simulink model "servo_20230915"  (R2022a)
settings: Solver=ode45  StartTime=0.0  StopTime=5  RelTol=1e-3
model workspace (MAT data in the model file):
  J = 0.0095
  Kt = 1
  La = 0.00097
  Ra = 0.11
values from neighbouring files (symbols this model uses):
  fe = 0.008    [para_for_math_pmsm.m]
  flux = 0.1827    [para_for_math_pmsm.m]
  Je = 0.003    [para_for_math_pmsm.m]
  Ld = 5.25e-3    (= 0.00525)    [para_for_math_pmsm.m]
  Lq = 5.25e-3    (= 0.00525)    [para_for_math_pmsm.m]
  Pn = 4    [para_for_math_pmsm.m]
  R = 0.299    [init_dc_servo.m]    (also in para_for_math_pmsm.m = 0.958)
undefined symbols (not defined in the file or in its folder): smiData, X, Y, Z
libraries: sm_lib x30, nesl_utility x16, spspowerguiLib x1
settings Model: ParameterArgumentNames=La,Ra  Creator=ccaao  LastModifiedBy=ccaao

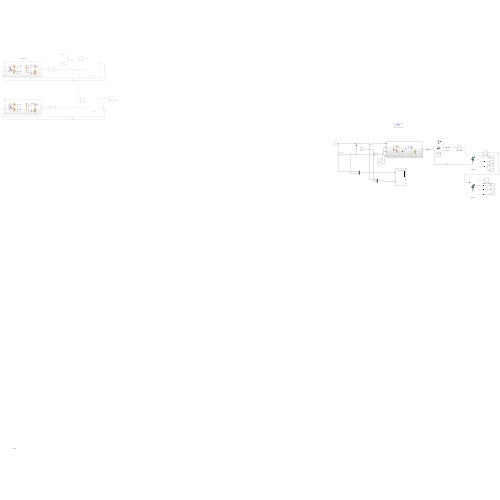
[thumbnail: Simulink's stored preview of the top-level diagram]
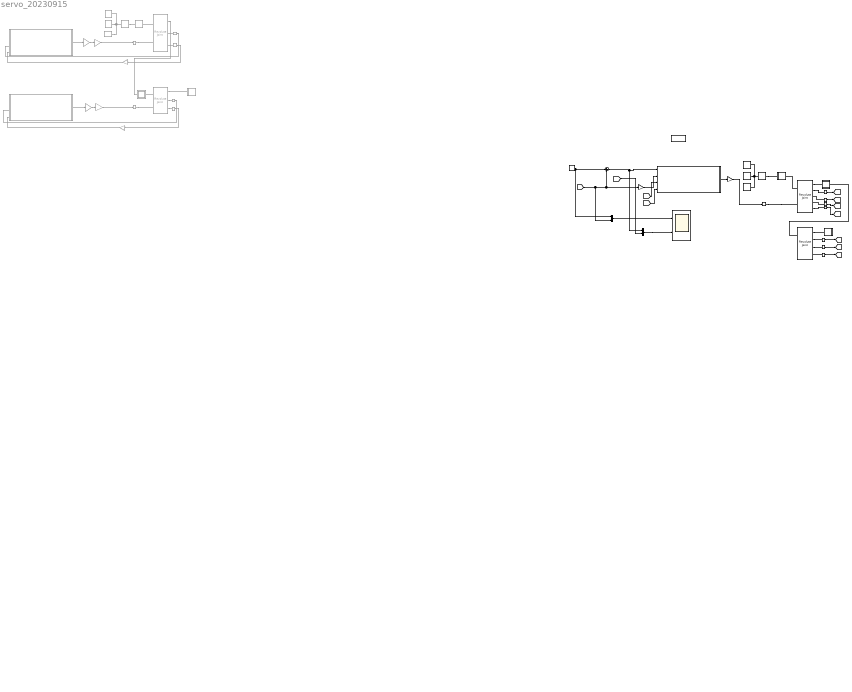
== system servo_20230915 ==
  note: position
  note: 电机方程
  Constant : Constant  Value=10
  Gain : Gain  Commented=on
  Gain1 : Gain  Commented=on  Gain=0.95
  Gain2 : Gain  Commented=on
  Gain3 : Gain  Commented=on  Gain=0.95
  Gain4 : Gain  Commented=on  Gain=Pn
  Gain5 : Gain  Commented=on  Gain=Pn
  Gain6 : Gain  Gain=Pn
  Gain8 : Gain  Gain=0.95
  MechanismConfiguration : sm_lib/Utilities/Mechanism Configuration  Commented=on  UniformGravity=Constant  GravityVector=[0 -9.80665 0]  GravityUnits=m/s^2  LinearizationDelta=0.001  JointModeTransitionNonlinearIterations=2
  MechanismConfiguration1 : sm_lib/Utilities/Mechanism Configuration  UniformGravity=Constant  GravityVector=[0 0 0]  GravityUnits=m/s^2  LinearizationDelta=0.001  JointModeTransitionNonlinearIterations=2
  Mux : Mux  Inputs=2
  Mux1 : Mux  Inputs=2
  PS-Simulink Converter{,1..3} (4 alike) : nesl_utility/PS-Simulink Converter  Commented=on  PhysicalDomain=network_engine_domain  SubClassName=ps_output  LeftPortType=input  RightPortType=output  PseudoPeriodic=off  Frequencies=[]  VectorFormat=inherit  Unit=inherit  AffineConversion=off
      settings: SourceProductBaseCode=SS,PW,VE
  PS-Simulink Converter10 : nesl_utility/PS-Simulink Converter  PhysicalDomain=network_engine_domain  SubClassName=ps_output  LeftPortType=input  RightPortType=output  PseudoPeriodic=off  Frequencies=[]  VectorFormat=1-D array  Unit=inherit  AffineConversion=off
      settings: SourceProductBaseCode=SS,PW,VE
  PS-Simulink Converter4 : nesl_utility/PS-Simulink Converter  PhysicalDomain=network_engine_domain  SubClassName=ps_output  LeftPortType=input  RightPortType=output  PseudoPeriodic=off  Frequencies=[]  VectorFormat=1-D array  Unit=rad  AffineConversion=off
      settings: SourceProductBaseCode=SS,PW,VE
  PS-Simulink Converter5 : nesl_utility/PS-Simulink Converter  PhysicalDomain=network_engine_domain  SubClassName=ps_output  LeftPortType=input  RightPortType=output  PseudoPeriodic=off  Frequencies=[]  VectorFormat=1-D array  Unit=N*m  AffineConversion=off
      settings: SourceProductBaseCode=SS,PW,VE
  PS-Simulink Converter6 : nesl_utility/PS-Simulink Converter  PhysicalDomain=network_engine_domain  SubClassName=ps_output  LeftPortType=input  RightPortType=output  PseudoPeriodic=off  Frequencies=[]  VectorFormat=1-D array  Unit=rad/s  AffineConversion=off
      settings: SourceProductBaseCode=SS,PW,VE
  PS-Simulink Converter7 : nesl_utility/PS-Simulink Converter  PhysicalDomain=network_engine_domain  SubClassName=ps_output  LeftPortType=input  RightPortType=output  PseudoPeriodic=off  Frequencies=[]  VectorFormat=1-D array  Unit=N*m  AffineConversion=off
      settings: SourceProductBaseCode=SS,PW,VE
  PS-Simulink Converter8 : nesl_utility/PS-Simulink Converter  PhysicalDomain=network_engine_domain  SubClassName=ps_output  LeftPortType=input  RightPortType=output  PseudoPeriodic=off  Frequencies=[]  VectorFormat=1-D array  Unit=rad  AffineConversion=off
      settings: SourceProductBaseCode=SS,PW,VE
  PS-Simulink Converter9 : nesl_utility/PS-Simulink Converter  PhysicalDomain=network_engine_domain  SubClassName=ps_output  LeftPortType=input  RightPortType=output  PseudoPeriodic=off  Frequencies=[]  VectorFormat=1-D array  Unit=rad/s  AffineConversion=off
      settings: SourceProductBaseCode=SS,PW,VE
  Revolute : sm_lib/Joints/Revolute Joint  Commented=on  JointMode=Normal  SenseConstraintForce=off  SenseConstraintForceX=off  SenseConstraintForceY=off  SenseConstraintForceZ=off  SenseConstraintTorque=off  SenseConstraintTorqueX=off  SenseConstraintTorqueY=off  SenseConstraintTorqueZ=off  SenseTotalForce=off  SenseTotalForceX=off  SenseTotalForceY=off  SenseTotalForceZ=off  SenseTotalTorque=off  SenseTotalTorqueX=off  SenseTotalTorqueY=off  SenseTotalTorqueZ=off  CompositeWrenchDir=FollowerOnBase  CompositeWrenchFrame=BaseFrame  EquilibriumPosition=0  EquilibriumPositionUnits=rad  SpringStiffness=0  SpringStiffnessUnits=N*m/rad  DampingCoefficient=0  DampingCoefficientUnits=N*m/(rad/s)  TorqueActuationMode=InputTorque  MotionActuationMode=ComputedMotion  SensePosition=on  SenseVelocity=on  SenseAcceleration=off  SenseTorqueForce=off  SenseLowerLimitTorqueForce=off  SenseUpperLimitTorqueForce=off  LowerLimitSpecify=off  LowerLimitBound=-90  LowerLimitBoundUnits=deg  LowerLimitStiffness=1e4  LowerLimitStiffnessUnits=N*m/deg  LowerLimitDamping=10  LowerLimitDampingUnits=N*m/(deg/s)  LowerLimitTransitionRegionWidth=0.1  LowerLimitTransitionRegionWidthUnits=deg  UpperLimitSpecify=off  UpperLimitBound=90  UpperLimitBoundUnits=deg  UpperLimitStiffness=1e4  UpperLimitStiffnessUnits=N*m/deg  UpperLimitDamping=10  UpperLimitDampingUnits=N*m/(deg/s)  UpperLimitTransitionRegionWidth=0.1  UpperLimitTransitionRegionWidthUnits=deg  PositionTargetSpecify=on  PositionTargetPriority=High  PositionTargetValue=smiData.RevoluteJoint(1).Rz.Pos  PositionTargetValueUnits=deg  VelocityTargetSpecify=on  VelocityTargetPriority=High  VelocityTargetValue=0  VelocityTargetValueUnits=rad/s
  Revolute1 : sm_lib/Joints/Revolute Joint  Commented=on  JointMode=Normal  SenseConstraintForce=off  SenseConstraintForceX=off  SenseConstraintForceY=off  SenseConstraintForceZ=off  SenseConstraintTorque=off  SenseConstraintTorqueX=off  SenseConstraintTorqueY=off  SenseConstraintTorqueZ=off  SenseTotalForce=off  SenseTotalForceX=off  SenseTotalForceY=off  SenseTotalForceZ=off  SenseTotalTorque=off  SenseTotalTorqueX=off  SenseTotalTorqueY=off  SenseTotalTorqueZ=off  CompositeWrenchDir=FollowerOnBase  CompositeWrenchFrame=BaseFrame  EquilibriumPosition=0  EquilibriumPositionUnits=rad  SpringStiffness=0  SpringStiffnessUnits=N*m/rad  DampingCoefficient=0  DampingCoefficientUnits=N*m/(rad/s)  TorqueActuationMode=InputTorque  MotionActuationMode=ComputedMotion  SensePosition=on  SenseVelocity=on  SenseAcceleration=off  SenseTorqueForce=off  SenseLowerLimitTorqueForce=off  SenseUpperLimitTorqueForce=off  LowerLimitSpecify=off  LowerLimitBound=-90  LowerLimitBoundUnits=deg  LowerLimitStiffness=1e4  LowerLimitStiffnessUnits=N*m/deg  LowerLimitDamping=10  LowerLimitDampingUnits=N*m/(deg/s)  LowerLimitTransitionRegionWidth=0.1  LowerLimitTransitionRegionWidthUnits=deg  UpperLimitSpecify=off  UpperLimitBound=90  UpperLimitBoundUnits=deg  UpperLimitStiffness=1e4  UpperLimitStiffnessUnits=N*m/deg  UpperLimitDamping=10  UpperLimitDampingUnits=N*m/(deg/s)  UpperLimitTransitionRegionWidth=0.1  UpperLimitTransitionRegionWidthUnits=deg  PositionTargetSpecify=on  PositionTargetPriority=High  PositionTargetValue=smiData.RevoluteJoint(2).Rz.Pos  PositionTargetValueUnits=deg  VelocityTargetSpecify=on  VelocityTargetPriority=High  VelocityTargetValue=0  VelocityTargetValueUnits=rad/s
  Revolute2 : sm_lib/Joints/Revolute Joint  JointMode=Normal  SenseConstraintForce=off  SenseConstraintForceX=off  SenseConstraintForceY=off  SenseConstraintForceZ=off  SenseConstraintTorque=off  SenseConstraintTorqueX=off  SenseConstraintTorqueY=off  SenseConstraintTorqueZ=off  SenseTotalForce=off  SenseTotalForceX=off  SenseTotalForceY=off  SenseTotalForceZ=off  SenseTotalTorque=off  SenseTotalTorqueX=off  SenseTotalTorqueY=off  SenseTotalTorqueZ=off  CompositeWrenchDir=FollowerOnBase  CompositeWrenchFrame=BaseFrame  EquilibriumPosition=0  EquilibriumPositionUnits=rad  SpringStiffness=0  SpringStiffnessUnits=N*m/rad  DampingCoefficient=0.0001  DampingCoefficientUnits=N*m/(rad/s)  TorqueActuationMode=InputTorque  MotionActuationMode=ComputedMotion  SensePosition=on  SenseVelocity=on  SenseAcceleration=on  SenseTorqueForce=on  SenseLowerLimitTorqueForce=off  SenseUpperLimitTorqueForce=off  LowerLimitSpecify=off  LowerLimitBound=-90  LowerLimitBoundUnits=deg  LowerLimitStiffness=1e4  LowerLimitStiffnessUnits=N*m/deg  LowerLimitDamping=10  LowerLimitDampingUnits=N*m/(deg/s)  LowerLimitTransitionRegionWidth=0.1  LowerLimitTransitionRegionWidthUnits=deg  UpperLimitSpecify=off  UpperLimitBound=90  UpperLimitBoundUnits=deg  UpperLimitStiffness=1e4  UpperLimitStiffnessUnits=N*m/deg  UpperLimitDamping=10  UpperLimitDampingUnits=N*m/(deg/s)  UpperLimitTransitionRegionWidth=0.1  UpperLimitTransitionRegionWidthUnits=deg  PositionTargetSpecify=off  PositionTargetPriority=High  PositionTargetValue=smiData.RevoluteJoint(1).Rz.Pos  PositionTargetValueUnits=deg  VelocityTargetSpecify=on  VelocityTargetPriority=High  VelocityTargetValue=0  VelocityTargetValueUnits=rad/s
  Revolute3 : sm_lib/Joints/Revolute Joint  JointMode=Normal  SenseConstraintForce=off  SenseConstraintForceX=off  SenseConstraintForceY=off  SenseConstraintForceZ=off  SenseConstraintTorque=off  SenseConstraintTorqueX=off  SenseConstraintTorqueY=off  SenseConstraintTorqueZ=off  SenseTotalForce=off  SenseTotalForceX=off  SenseTotalForceY=off  SenseTotalForceZ=off  SenseTotalTorque=off  SenseTotalTorqueX=off  SenseTotalTorqueY=off  SenseTotalTorqueZ=off  CompositeWrenchDir=FollowerOnBase  CompositeWrenchFrame=BaseFrame  EquilibriumPosition=0  EquilibriumPositionUnits=rad  SpringStiffness=1000  SpringStiffnessUnits=N*m/rad  DampingCoefficient=0.0001  DampingCoefficientUnits=N*m/(rad/s)  TorqueActuationMode=InputTorque  MotionActuationMode=ComputedMotion  SensePosition=on  SenseVelocity=on  SenseAcceleration=off  SenseTorqueForce=on  SenseLowerLimitTorqueForce=off  SenseUpperLimitTorqueForce=off  LowerLimitSpecify=on  LowerLimitBound=40  LowerLimitBoundUnits=deg  LowerLimitStiffness=1e7  LowerLimitStiffnessUnits=N*m/deg  LowerLimitDamping=10  LowerLimitDampingUnits=N*m/(deg/s)  LowerLimitTransitionRegionWidth=100  LowerLimitTransitionRegionWidthUnits=deg  UpperLimitSpecify=on  UpperLimitBound=120  UpperLimitBoundUnits=deg  UpperLimitStiffness=1e7  UpperLimitStiffnessUnits=N*m/deg  UpperLimitDamping=10  UpperLimitDampingUnits=N*m/(deg/s)  UpperLimitTransitionRegionWidth=100  UpperLimitTransitionRegionWidthUnits=deg  PositionTargetSpecify=on  PositionTargetPriority=Low  PositionTargetValue=80  PositionTargetValueUnits=deg  VelocityTargetSpecify=on  VelocityTargetPriority=High  VelocityTargetValue=0  VelocityTargetValueUnits=rad/s
  Scope : Scope  NumInputPorts=2
  Simulink-PS Converter : nesl_utility/Simulink-PS Converter  Commented=on  PhysicalDomain=network_engine_domain  SubClassName=ps_input  LeftPortType=input  RightPortType=output  PseudoPeriodic=off  Frequencies=[]  NoiseDistribution=none  NoiseParameters=[]  Unit=1  AffineConversion=off  FilteringAndDerivatives=provide  SimscapeFilterOrder=1  InputFilterTimeConstant=0.001  UdotUserProvided=0
      settings: SourceProductBaseCode=SS,PW,VE
  Simulink-PS Converter1 : nesl_utility/Simulink-PS Converter  Commented=on  PhysicalDomain=network_engine_domain  SubClassName=ps_input  LeftPortType=input  RightPortType=output  PseudoPeriodic=off  Frequencies=[]  NoiseDistribution=none  NoiseParameters=[]  Unit=1  AffineConversion=off  FilteringAndDerivatives=provide  SimscapeFilterOrder=1  InputFilterTimeConstant=0.001  UdotUserProvided=0
      settings: SourceProductBaseCode=SS,PW,VE
  Simulink-PS Converter2 : nesl_utility/Simulink-PS Converter  PhysicalDomain=network_engine_domain  SubClassName=ps_input  LeftPortType=input  RightPortType=output  PseudoPeriodic=off  Frequencies=[]  NoiseDistribution=none  NoiseParameters=[]  Unit=1  AffineConversion=off  FilteringAndDerivatives=provide  SimscapeFilterOrder=1  InputFilterTimeConstant=0.001  UdotUserProvided=0
      settings: SourceProductBaseCode=SS,PW,VE
  Solver Configuration : nesl_utility/Solver Configuration  Commented=on  PhysicalDomain=network_engine_domain  SubClassName=solver  LeftPortType=input  RightPortType=generic  Tones=[]  Harmonics=[]  SimulateNoise=off  Profile=off  UseLocalSampling=off  EnableSwitchedLinearOptims=on  FrequencyDomain=off  UseCCode=off  RelTol=0.001  AbsTol=0.001  MinStep=1e-09  ToWorkspace=off  RevertToSquareIcSolve=off  NumHomotopyIterations=100  PhasorMode=off  PhasorModeNumHarmonics=1  IndexReductionMethod=DerivativeReplacement  DoDC=off  ResidualTolerance=1e-09  UseLocalSolver=off  LocalSolverChoice=NE_BACKWARD_EULER_ADVANCER  LocalSolverSampleTime=0.001  DoFixedCost=off  MaxNonlinIter=3  MaxModeIter=2  ComputeImpulses=off  ImpulseIterations=2  LinearAlgebra=auto  LinearAlgebraNumThread=0  EquationFormulation=NE_TIME_EF  DelaysMemoryBudget=1024  AutomaticFiltering=on  FilteringTimeConstant=0.001  PartitionStorageMethod=AS_NEEDED  PartitionMemoryBudget=1024  PartitionMethod=ROBUST
      settings: SourceProductBaseCode=SS,PW,VE
  Solver Configuration1 : nesl_utility/Solver Configuration  PhysicalDomain=network_engine_domain  SubClassName=solver  LeftPortType=input  RightPortType=generic  Tones=[]  Harmonics=[]  SimulateNoise=off  Profile=off  UseLocalSampling=off  EnableSwitchedLinearOptims=on  FrequencyDomain=off  UseCCode=off  RelTol=0.001  AbsTol=1e-06  MinStep=1e-09  ToWorkspace=off  RevertToSquareIcSolve=off  NumHomotopyIterations=100  PhasorMode=off  PhasorModeNumHarmonics=1  IndexReductionMethod=DerivativeReplacement  DoDC=off  ResidualTolerance=1e-09  UseLocalSolver=off  LocalSolverChoice=NE_BACKWARD_EULER_ADVANCER  LocalSolverSampleTime=0.001  DoFixedCost=off  MaxNonlinIter=3  MaxModeIter=2  ComputeImpulses=off  ImpulseIterations=2  LinearAlgebra=Sparse  LinearAlgebraNumThread=0  EquationFormulation=NE_TIME_EF  DelaysMemoryBudget=1024  AutomaticFiltering=on  FilteringTimeConstant=0.001  PartitionStorageMethod=AS_NEEDED  PartitionMemoryBudget=1024  PartitionMethod=FAST
      settings: SourceProductBaseCode=SS,PW,VE
  Subsystem1 : Subsystem  Commented=on
  Subsystem2 : Subsystem  Commented=on
  Subsystem3 : Subsystem
  Sum : Sum  Inputs=|+-
  Transform : sm_lib/Frames and Transforms/Rigid Transform  Commented=on  TranslationMethod=Cartesian  TranslationStandardOffset=0  TranslationLengthUnit=mm  TranslationStandardAxis=+Z  TranslationCartesianOffset=smiData.RigidTransform(5).translation  TranslationROffset=0  TranslationROffsetUnits=m  TranslationZOffset=0  TranslationZOffsetUnits=m  TranslationThetaOffset=0  TranslationThetaOffsetUnits=deg  RotationMethod=ArbitraryAxis  RotationAngleUnits=rad  RotationStandardAxis=+Z  RotationAngle=smiData.RigidTransform(5).angle  RotationArbitraryAxis=smiData.RigidTransform(5).axis  FollAlignAxisA=+X  BaseAlignAxisA=+Y  FollAlignAxisB=+Y  BaseAlignAxisB=+Z  RotationSequenceAxes=FollowerAxes  RotationSequence=XYX  RotationSequenceAngles=[0 0 0]  RotationSequenceAnglesUnits=deg  RotationMatrix=[1 0 0; 0 1 0; 0 0 1]
  Transform1 : sm_lib/Frames and Transforms/Rigid Transform  TranslationMethod=Cartesian  TranslationStandardOffset=0  TranslationLengthUnit=mm  TranslationStandardAxis=+Z  TranslationCartesianOffset=smiData.RigidTransform(5).translation  TranslationROffset=0  TranslationROffsetUnits=m  TranslationZOffset=0  TranslationZOffsetUnits=m  TranslationThetaOffset=0  TranslationThetaOffsetUnits=deg  RotationMethod=ArbitraryAxis  RotationAngleUnits=rad  RotationStandardAxis=+Z  RotationAngle=smiData.RigidTransform(5).angle  RotationArbitraryAxis=smiData.RigidTransform(5).axis  FollAlignAxisA=+X  BaseAlignAxisA=+Y  FollAlignAxisB=+Y  BaseAlignAxisB=+Z  RotationSequenceAxes=FollowerAxes  RotationSequence=XYX  RotationSequenceAngles=[0 0 0]  RotationSequenceAnglesUnits=deg  RotationMatrix=[1 0 0; 0 1 0; 0 0 1]
  World : sm_lib/Frames and Transforms/World Frame  Commented=on
  World1 : sm_lib/Frames and Transforms/World Frame
  diban_1_RIGID : Subsystem  Commented=on
  diban_1_RIGID1 : Subsystem
  hengliang1_1_RIGID : Subsystem  Commented=on
  hengliang1_1_RIGID1 : Subsystem
  jijia_1_RIGID : Subsystem  Commented=on
  jijia_1_RIGID1 : Subsystem
  powergui : spspowerguiLib/powergui  Priority=1  SimulationMode=Discrete  SampleTime=50e-5  frequency=60  Iterations=50  frequencyindice=60  Pbase=100e6  ErrMax=1e-4  UnitsV=kV  UnitsW=MW  buscounter=0  FunctionMessages=off  echomessages=off  EnableUseOfTLC=off  CurrentSourceSwitches=off  DisableSnubberDevices=off  DisableRonSwitches=off  DisableVfSwitches=off  DisplayEquations=off  AutomaticDiscreteSolvers=off  SolverType=Tustin/Backward Euler (TBE)  Interpol=off  ExternalGateDelay=off  methode=off  Ts=100  x0status=blocks  SPID=on  SwTol=0  HookPort=off  NonlinearTolerance=1e-4  nMaxIteration=100  ContinueOnMaxIteration=off  RestoreLinks=warning  ResistiveCurrentMeasurement=off  Frange=[0:2:500]  Ylog=off  Xlog=on  ShowGrid=off  save=off  variable=ZData  structure=0  ZoomFFT=off  StartTime=0.0  cycles=1  DisplayStyle=1  fundamental=60  FreqAxis=off  MaxFrequency=1000  frequencyindicesteady=1  RmsSteady=1  display=off
  tag scope: a1=global, q1=global, q2=global, t1=global, t2=global, w1=global, w2=global
  wires:
  Subsystem1/1(Tm) -> Gain/1
  Gain/1 -> Gain1/1
  Gain1/1 -> Simulink-PS Converter/1
  PS-Simulink Converter/1 -> Subsystem1/3(theta)
  PS-Simulink Converter1/1 -> Gain5/1
  Gain3/1 -> Simulink-PS Converter1/1
  Gain2/1 -> Gain3/1
  Subsystem2/1(Tm) -> Gain2/1
  PS-Simulink Converter2/1 -> Subsystem2/3(theta)
  PS-Simulink Converter3/1 -> Gain4/1
  Gain4/1 -> Subsystem2/4(we)
  Gain5/1 -> Subsystem1/4(we)
  Sum/1 -> Subsystem3/1(uq), Mux1/1
  PS-Simulink Converter7/1 -> [t2]
  PS-Simulink Converter5/1 -> [t1]
  PS-Simulink Converter4/1 -> [q1]
  PS-Simulink Converter9/1 -> [w2]
  PS-Simulink Converter6/1 -> [w1]
  PS-Simulink Converter8/1 -> [q2]
  Constant/1 -> Sum/1, Mux/1
  Gain6/1 -> Subsystem3/2(we)
  [w1] -> Sum/2, Gain6/1, Mux/2
  [t1] -> Mux1/2
  Subsystem3/1(Tm) -> Gain8/1
  Gain8/1 -> Simulink-PS Converter2/1
  Mux/1 -> Scope/1
  Mux1/1 -> Scope/2
  PS-Simulink Converter10/1 -> [a1]
  [a1] -> Subsystem3/3(Input)
  [w1] -> Subsystem3/4(Input1)
  connections:
  MechanismConfiguration/RConn1 -- Transform/LConn1 -- World/RConn1 -- Solver Configuration/RConn1
  Revolute1/RConn1 -- hengliang1_1_RIGID/LConn1
  Transform/RConn1 -- jijia_1_RIGID/LConn1
  Revolute/RConn1 -- diban_1_RIGID/LConn1
  Revolute/LConn1 -- jijia_1_RIGID/RConn1
  Revolute1/LConn1 -- diban_1_RIGID/RConn1
  Simulink-PS Converter/RConn1 -- Revolute/LConn2
  PS-Simulink Converter/LConn1 -- Revolute/RConn2
  PS-Simulink Converter1/LConn1 -- Revolute/RConn3
  Simulink-PS Converter1/RConn1 -- Revolute1/LConn2
  Revolute1/RConn2 -- PS-Simulink Converter2/LConn1
  Revolute1/RConn3 -- PS-Simulink Converter3/LConn1
  Revolute2/RConn2 -- PS-Simulink Converter4/LConn1
  Revolute3/RConn2 -- PS-Simulink Converter8/LConn1
  Revolute3/RConn3 -- PS-Simulink Converter9/LConn1
  World1/RConn1 -- MechanismConfiguration1/RConn1 -- Solver Configuration1/RConn1 -- Transform1/LConn1
  Revolute3/RConn1 -- hengliang1_1_RIGID1/LConn1
  Revolute2/RConn5 -- PS-Simulink Converter5/LConn1
  Simulink-PS Converter2/RConn1 -- Revolute2/LConn2
  PS-Simulink Converter6/LConn1 -- Revolute2/RConn3
  Revolute2/LConn1 -- jijia_1_RIGID1/RConn1
  Transform1/RConn1 -- jijia_1_RIGID1/LConn1
  PS-Simulink Converter7/LConn1 -- Revolute3/RConn4
  Revolute2/RConn1 -- diban_1_RIGID1/LConn1
  Revolute3/LConn1 -- diban_1_RIGID1/RConn1
  PS-Simulink Converter10/LConn1 -- Revolute2/RConn4

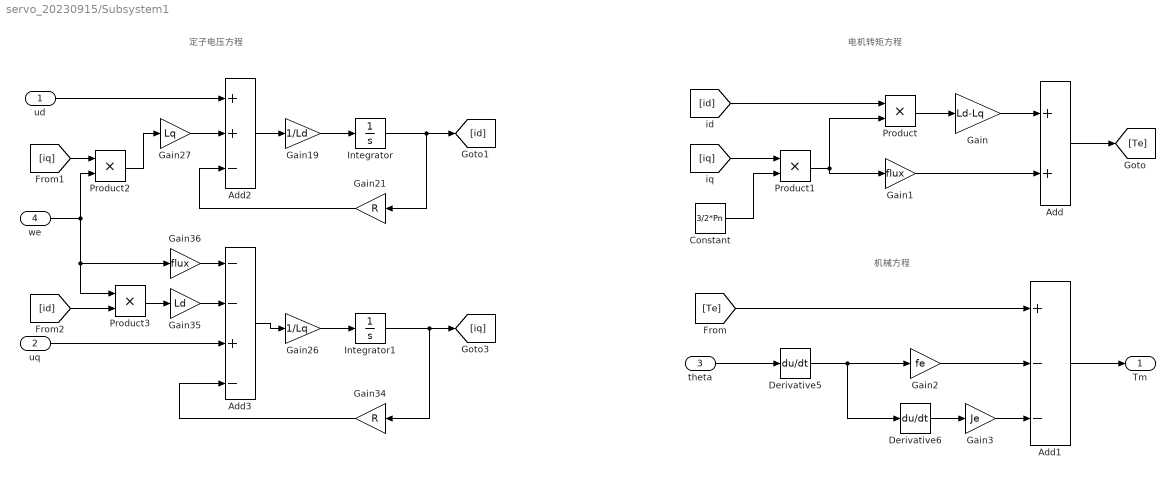
== system servo_20230915/Subsystem1 ==
  note: 电机转矩方程
  note: 机械方程
  note: 定子电压方程
  ud : Inport
  uq : Inport  Port=2
  theta : Inport  Port=3
  we : Inport  Port=4
  Add : Sum
  Add1 : Sum  Inputs=+--
  Add2 : Sum  Inputs=++-
  Add3 : Sum  Inputs=--+-
  Constant : Constant  Value=3/2*Pn
  Derivative5 : Derivative
  Derivative6 : Derivative
  Gain : Gain  Gain=Ld-Lq
  Gain1 : Gain  Gain=flux
  Gain19 : Gain  Gain=1/Ld
  Gain2 : Gain  Gain=fe
  Gain21 : Gain  Gain=R
  Gain26 : Gain  Gain=1/Lq
  Gain27 : Gain  Gain=Lq
  Gain3 : Gain  Gain=Je
  Gain34 : Gain  Gain=R
  Gain35 : Gain  Gain=Ld
  Gain36 : Gain  Gain=flux
  Integrator : Integrator
  Integrator1 : Integrator
  Product{,1..3} (4 alike) : Product
  Tm : Outport
  wires:
  [id] -> Product3/2
  Add1/1 -> Tm/1
  [iq] -> Product1/1
  Gain19/1 -> Integrator/1
  theta/1 -> Derivative5/1
  Integrator/1 -> Gain21/1, [id]
  [Te] -> Add1/1
  Gain26/1 -> Integrator1/1
  [id] -> Product/1
  Product3/1 -> Gain35/1
  Gain34/1 -> Add3/4
  Gain1/1 -> Add/2
  Add3/1 -> Gain26/1
  Constant/1 -> Product1/2
  Add/1 -> [Te]
  Gain/1 -> Add/1
  we/1 -> Gain36/1, Product3/1, Product2/2
  Derivative6/1 -> Gain3/1
  Integrator1/1 -> Gain34/1, [iq]
  Derivative5/1 -> Derivative6/1, Gain2/1
  Gain3/1 -> Add1/3
  ud/1 -> Add2/1
  [iq] -> Product2/1
  Gain21/1 -> Add2/3
  Gain2/1 -> Add1/2
  Gain27/1 -> Add2/2
  uq/1 -> Add3/3
  Product2/1 -> Gain27/1
  Gain35/1 -> Add3/2
  Product/1 -> Gain/1
  Gain36/1 -> Add3/1
  Product1/1 -> Product/2, Gain1/1
  Add2/1 -> Gain19/1

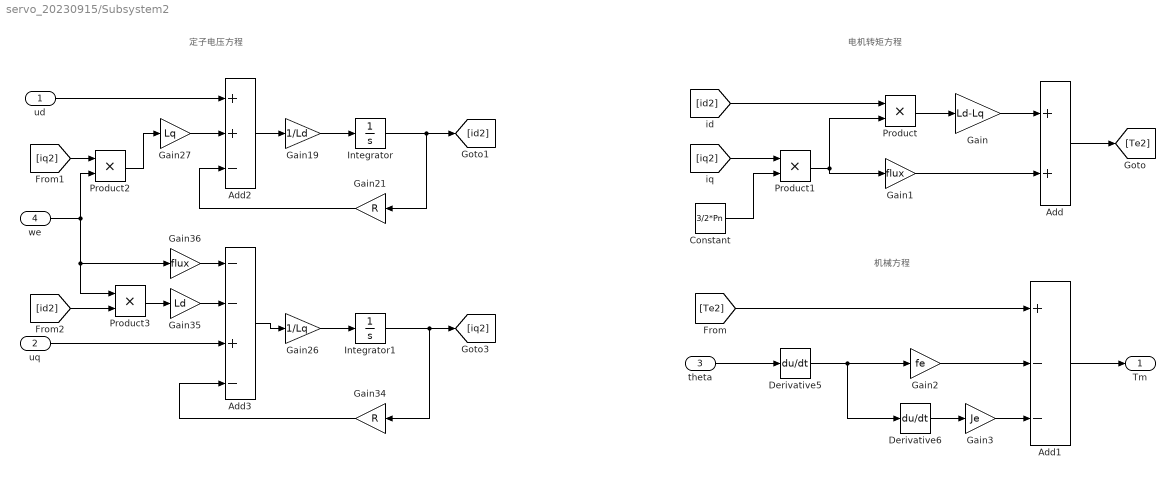
== system servo_20230915/Subsystem2 ==
  note: 定子电压方程
  note: 机械方程
  note: 电机转矩方程
  ud : Inport
  uq : Inport  Port=2
  theta : Inport  Port=3
  we : Inport  Port=4
  Add : Sum
  Add1 : Sum  Inputs=+--
  Add2 : Sum  Inputs=++-
  Add3 : Sum  Inputs=--+-
  Constant : Constant  Value=3/2*Pn
  Derivative5 : Derivative
  Derivative6 : Derivative
  Gain : Gain  Gain=Ld-Lq
  Gain1 : Gain  Gain=flux
  Gain19 : Gain  Gain=1/Ld
  Gain2 : Gain  Gain=fe
  Gain21 : Gain  Gain=R
  Gain26 : Gain  Gain=1/Lq
  Gain27 : Gain  Gain=Lq
  Gain3 : Gain  Gain=Je
  Gain34 : Gain  Gain=R
  Gain35 : Gain  Gain=Ld
  Gain36 : Gain  Gain=flux
  Integrator : Integrator
  Integrator1 : Integrator
  Product{,1..3} (4 alike) : Product
  Tm : Outport
  wires:
  Add2/1 -> Gain19/1
  Product1/1 -> Gain1/1, Product/2
  Gain36/1 -> Add3/1
  Product/1 -> Gain/1
  Gain35/1 -> Add3/2
  Product2/1 -> Gain27/1
  uq/1 -> Add3/3
  Gain27/1 -> Add2/2
  Gain2/1 -> Add1/2
  Gain21/1 -> Add2/3
  [iq2] -> Product2/1
  ud/1 -> Add2/1
  Gain3/1 -> Add1/3
  Derivative5/1 -> Gain2/1, Derivative6/1
  Integrator1/1 -> [iq2], Gain34/1
  Derivative6/1 -> Gain3/1
  we/1 -> Product2/2, Product3/1, Gain36/1
  Gain/1 -> Add/1
  Add/1 -> [Te2]
  Constant/1 -> Product1/2
  Add3/1 -> Gain26/1
  Gain1/1 -> Add/2
  Gain34/1 -> Add3/4
  Product3/1 -> Gain35/1
  [id2] -> Product/1
  Gain26/1 -> Integrator1/1
  [Te2] -> Add1/1
  Integrator/1 -> [id2], Gain21/1
  theta/1 -> Derivative5/1
  Gain19/1 -> Integrator/1
  [iq2] -> Product1/1
  Add1/1 -> Tm/1
  [id2] -> Product3/2

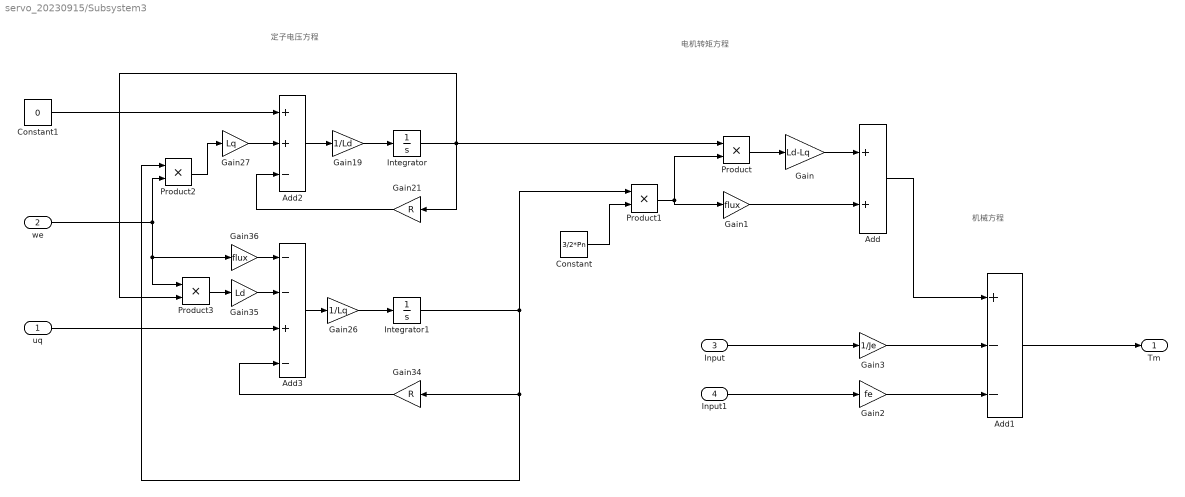
== system servo_20230915/Subsystem3 ==
  note: 定子电压方程
  note: 机械方程
  note: 电机转矩方程
  uq : Inport
  we : Inport  Port=2
  Input : Inport  Port=3
  Input1 : Inport  Port=4
  Add : Sum
  Add1 : Sum  Inputs=+--
  Add2 : Sum  Inputs=++-
  Add3 : Sum  Inputs=--+-
  Constant : Constant  Value=3/2*Pn
  Constant1 : Constant  Value=0
  Gain : Gain  Gain=Ld-Lq
  Gain1 : Gain  Gain=flux
  Gain19 : Gain  Gain=1/Ld
  Gain2 : Gain  Gain=fe
  Gain21 : Gain  Gain=R
  Gain26 : Gain  Gain=1/Lq
  Gain27 : Gain  Gain=Lq
  Gain3 : Gain  Gain=1/Je
  Gain34 : Gain  Gain=R
  Gain35 : Gain  Gain=Ld
  Gain36 : Gain  Gain=flux
  Integrator : Integrator
  Integrator1 : Integrator
  Product{,1..3} (4 alike) : Product
  Tm : Outport
  wires:
  Add2/1 -> Gain19/1
  Product1/1 -> Gain1/1, Product/2
  Gain36/1 -> Add3/1
  Product/1 -> Gain/1
  Gain35/1 -> Add3/2
  Product2/1 -> Gain27/1
  uq/1 -> Add3/3
  Gain27/1 -> Add2/2
  Gain21/1 -> Add2/3
  Integrator1/1 -> Product2/1, Gain34/1, Product1/1
  Constant1/1 -> Add2/1
  we/1 -> Product2/2, Product3/1, Gain36/1
  Gain/1 -> Add/1
  Constant/1 -> Product1/2
  Add3/1 -> Gain26/1
  Gain1/1 -> Add/2
  Gain34/1 -> Add3/4
  Product3/1 -> Gain35/1
  Gain26/1 -> Integrator1/1
  Add/1 -> Add1/1
  Gain19/1 -> Integrator/1
  Integrator/1 -> Gain21/1, Product3/2, Product/1
  Gain3/1 -> Add1/2
  Gain2/1 -> Add1/3
  Add1/1 -> Tm/1
  Input/1 -> Gain3/1
  Input1/1 -> Gain2/1

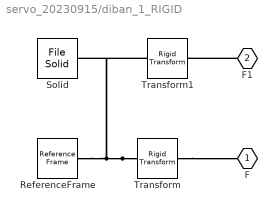
== system servo_20230915/diban_1_RIGID ==
  ReferenceFrame : sm_lib/Frames and Transforms/Reference Frame
  Solid : sm_lib/Body Elements/File Solid  ExtGeomFileName=diban_默认_sldprt.STEP  UnitType=FromFile  ExtGeomFileUnits=m  StepReaderType=HEX  ExportConvexHullGeometry=off  InertiaType=Custom  Mass=smiData.Solid(1).mass  MassUnits=kg  CenterOfMass=smiData.Solid(1).CoM  CenterOfMassUnits=mm  MomentsOfInertia=smiData.Solid(1).MoI  MomentsOfInertiaUnits=kg*mm^2  ProductsOfInertia=smiData.Solid(1).PoI  ProductsOfInertiaUnits=kg*mm^2  BasedOnType=Density  Density=1000  DensityUnits=kg/m^3  DoExposeReferenceFrame=on  SerializedFrames=<Frames/>  GraphicType=FromGeometry  MarkerShape=Sphere  MarkerSize=10  GraphicVisPropType=SimpleVisualProperties  GraphicDiffuseColor=smiData.Solid(1).color  GraphicSpecularColor=[0.5 0.5 0.5 1.0]  GraphicAmbientColor=[0.15 0.15 0.15 1.0]  GraphicEmissiveColor=[0.0 0.0 0.0 1.0]  GraphicShininess=75  GraphicOpacity=smiData.Solid(1).opacity
  Transform : sm_lib/Frames and Transforms/Rigid Transform  TranslationMethod=Cartesian  TranslationStandardOffset=0  TranslationLengthUnit=mm  TranslationStandardAxis=+Z  TranslationCartesianOffset=smiData.RigidTransform(2).translation  TranslationROffset=0  TranslationROffsetUnits=m  TranslationZOffset=0  TranslationZOffsetUnits=m  TranslationThetaOffset=0  TranslationThetaOffsetUnits=deg  RotationMethod=ArbitraryAxis  RotationAngleUnits=rad  RotationStandardAxis=+Z  RotationAngle=smiData.RigidTransform(2).angle  RotationArbitraryAxis=smiData.RigidTransform(2).axis  FollAlignAxisA=+X  BaseAlignAxisA=+Y  FollAlignAxisB=+Y  BaseAlignAxisB=+Z  RotationSequenceAxes=FollowerAxes  RotationSequence=XYX  RotationSequenceAngles=[0 0 0]  RotationSequenceAnglesUnits=deg  RotationMatrix=[1 0 0; 0 1 0; 0 0 1]
  Transform1 : sm_lib/Frames and Transforms/Rigid Transform  TranslationMethod=Cartesian  TranslationStandardOffset=0  TranslationLengthUnit=mm  TranslationStandardAxis=+Z  TranslationCartesianOffset=smiData.RigidTransform(3).translation  TranslationROffset=0  TranslationROffsetUnits=m  TranslationZOffset=0  TranslationZOffsetUnits=m  TranslationThetaOffset=0  TranslationThetaOffsetUnits=deg  RotationMethod=ArbitraryAxis  RotationAngleUnits=rad  RotationStandardAxis=+Z  RotationAngle=smiData.RigidTransform(3).angle  RotationArbitraryAxis=smiData.RigidTransform(3).axis  FollAlignAxisA=+X  BaseAlignAxisA=+Y  FollAlignAxisB=+Y  BaseAlignAxisB=+Z  RotationSequenceAxes=FollowerAxes  RotationSequence=XYX  RotationSequenceAngles=[0 0 0]  RotationSequenceAnglesUnits=deg  RotationMatrix=[1 0 0; 0 1 0; 0 0 1]
  F : PMIOPort  Side=Left
  F1 : PMIOPort  Port=2  Side=Right
  connections:
  Transform/LConn1 -- ReferenceFrame/RConn1 -- Solid/RConn1 -- Transform1/LConn1
  Transform/RConn1 -- F/RConn1
  F1/RConn1 -- Transform1/RConn1

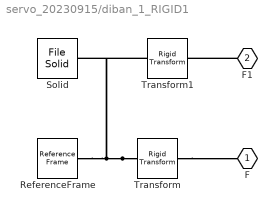
== system servo_20230915/diban_1_RIGID1 ==
  ReferenceFrame : sm_lib/Frames and Transforms/Reference Frame
  Solid : sm_lib/Body Elements/File Solid  ExtGeomFileName=diban_默认_sldprt.STEP  UnitType=FromFile  ExtGeomFileUnits=m  StepReaderType=HEX  ExportConvexHullGeometry=off  InertiaType=Custom  Mass=smiData.Solid(1).mass  MassUnits=kg  CenterOfMass=smiData.Solid(1).CoM  CenterOfMassUnits=mm  MomentsOfInertia=smiData.Solid(1).MoI  MomentsOfInertiaUnits=kg*mm^2  ProductsOfInertia=smiData.Solid(1).PoI  ProductsOfInertiaUnits=kg*mm^2  BasedOnType=Density  Density=1000  DensityUnits=kg/m^3  DoExposeReferenceFrame=on  SerializedFrames=<Frames/>  GraphicType=FromGeometry  MarkerShape=Sphere  MarkerSize=10  GraphicVisPropType=SimpleVisualProperties  GraphicDiffuseColor=[0.6 0.6 0.6]  GraphicSpecularColor=[0.5 0.5 0.5 1.0]  GraphicAmbientColor=[0.15 0.15 0.15 1.0]  GraphicEmissiveColor=[0.0 0.0 0.0 1.0]  GraphicShininess=75  GraphicOpacity=smiData.Solid(1).opacity
  Transform : sm_lib/Frames and Transforms/Rigid Transform  TranslationMethod=Cartesian  TranslationStandardOffset=0  TranslationLengthUnit=mm  TranslationStandardAxis=+Z  TranslationCartesianOffset=smiData.RigidTransform(2).translation  TranslationROffset=0  TranslationROffsetUnits=m  TranslationZOffset=0  TranslationZOffsetUnits=m  TranslationThetaOffset=0  TranslationThetaOffsetUnits=deg  RotationMethod=ArbitraryAxis  RotationAngleUnits=rad  RotationStandardAxis=+Z  RotationAngle=smiData.RigidTransform(2).angle  RotationArbitraryAxis=smiData.RigidTransform(2).axis  FollAlignAxisA=+X  BaseAlignAxisA=+Y  FollAlignAxisB=+Y  BaseAlignAxisB=+Z  RotationSequenceAxes=FollowerAxes  RotationSequence=XYX  RotationSequenceAngles=[0 0 0]  RotationSequenceAnglesUnits=deg  RotationMatrix=[1 0 0; 0 1 0; 0 0 1]
  Transform1 : sm_lib/Frames and Transforms/Rigid Transform  TranslationMethod=Cartesian  TranslationStandardOffset=0  TranslationLengthUnit=mm  TranslationStandardAxis=+Z  TranslationCartesianOffset=smiData.RigidTransform(3).translation  TranslationROffset=0  TranslationROffsetUnits=m  TranslationZOffset=0  TranslationZOffsetUnits=m  TranslationThetaOffset=0  TranslationThetaOffsetUnits=deg  RotationMethod=ArbitraryAxis  RotationAngleUnits=rad  RotationStandardAxis=+Z  RotationAngle=smiData.RigidTransform(3).angle  RotationArbitraryAxis=smiData.RigidTransform(3).axis  FollAlignAxisA=+X  BaseAlignAxisA=+Y  FollAlignAxisB=+Y  BaseAlignAxisB=+Z  RotationSequenceAxes=FollowerAxes  RotationSequence=XYX  RotationSequenceAngles=[0 0 0]  RotationSequenceAnglesUnits=deg  RotationMatrix=[1 0 0; 0 1 0; 0 0 1]
  F : PMIOPort  Side=Left
  F1 : PMIOPort  Port=2  Side=Right
  connections:
  Transform/LConn1 -- ReferenceFrame/RConn1 -- Solid/RConn1 -- Transform1/LConn1
  Transform/RConn1 -- F/RConn1
  F1/RConn1 -- Transform1/RConn1

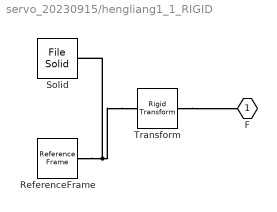
== system servo_20230915/hengliang1_1_RIGID ==
  ReferenceFrame : sm_lib/Frames and Transforms/Reference Frame
  Solid : sm_lib/Body Elements/File Solid  ExtGeomFileName=hengliang1_默认_sldprt.STEP  UnitType=FromFile  ExtGeomFileUnits=m  StepReaderType=HEX  ExportConvexHullGeometry=off  InertiaType=Custom  Mass=smiData.Solid(3).mass  MassUnits=kg  CenterOfMass=smiData.Solid(3).CoM  CenterOfMassUnits=mm  MomentsOfInertia=smiData.Solid(3).MoI  MomentsOfInertiaUnits=kg*mm^2  ProductsOfInertia=smiData.Solid(3).PoI  ProductsOfInertiaUnits=kg*mm^2  BasedOnType=Density  Density=1000  DensityUnits=kg/m^3  DoExposeReferenceFrame=on  SerializedFrames=<Frames/>  GraphicType=FromGeometry  MarkerShape=Sphere  MarkerSize=10  GraphicVisPropType=SimpleVisualProperties  GraphicDiffuseColor=smiData.Solid(3).color  GraphicSpecularColor=[0.5 0.5 0.5 1.0]  GraphicAmbientColor=[0.15 0.15 0.15 1.0]  GraphicEmissiveColor=[0.0 0.0 0.0 1.0]  GraphicShininess=75  GraphicOpacity=smiData.Solid(3).opacity
  Transform : sm_lib/Frames and Transforms/Rigid Transform  TranslationMethod=Cartesian  TranslationStandardOffset=0  TranslationLengthUnit=mm  TranslationStandardAxis=+Z  TranslationCartesianOffset=smiData.RigidTransform(4).translation  TranslationROffset=0  TranslationROffsetUnits=m  TranslationZOffset=0  TranslationZOffsetUnits=m  TranslationThetaOffset=0  TranslationThetaOffsetUnits=deg  RotationMethod=ArbitraryAxis  RotationAngleUnits=rad  RotationStandardAxis=+Z  RotationAngle=smiData.RigidTransform(4).angle  RotationArbitraryAxis=smiData.RigidTransform(4).axis  FollAlignAxisA=+X  BaseAlignAxisA=+Y  FollAlignAxisB=+Y  BaseAlignAxisB=+Z  RotationSequenceAxes=FollowerAxes  RotationSequence=XYX  RotationSequenceAngles=[0 0 0]  RotationSequenceAnglesUnits=deg  RotationMatrix=[1 0 0; 0 1 0; 0 0 1]
  F : PMIOPort  Side=Left
  connections:
  Transform/RConn1 -- F/RConn1
  Transform/LConn1 -- ReferenceFrame/RConn1 -- Solid/RConn1

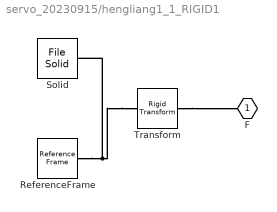
== system servo_20230915/hengliang1_1_RIGID1 ==
  ReferenceFrame : sm_lib/Frames and Transforms/Reference Frame
  Solid : sm_lib/Body Elements/File Solid  ExtGeomFileName=hengliang1_默认_sldprt.STEP  UnitType=FromFile  ExtGeomFileUnits=m  StepReaderType=HEX  ExportConvexHullGeometry=off  InertiaType=Custom  Mass=smiData.Solid(3).mass  MassUnits=kg  CenterOfMass=smiData.Solid(3).CoM  CenterOfMassUnits=mm  MomentsOfInertia=smiData.Solid(3).MoI  MomentsOfInertiaUnits=kg*mm^2  ProductsOfInertia=smiData.Solid(3).PoI  ProductsOfInertiaUnits=kg*mm^2  BasedOnType=Density  Density=1000  DensityUnits=kg/m^3  DoExposeReferenceFrame=on  SerializedFrames=<Frames/>  GraphicType=FromGeometry  MarkerShape=Sphere  MarkerSize=10  GraphicVisPropType=SimpleVisualProperties  GraphicDiffuseColor=smiData.Solid(3).color  GraphicSpecularColor=[0.5 0.5 0.5 1.0]  GraphicAmbientColor=[0.15 0.15 0.15 1.0]  GraphicEmissiveColor=[0.0 0.0 0.0 1.0]  GraphicShininess=75  GraphicOpacity=smiData.Solid(3).opacity
  Transform : sm_lib/Frames and Transforms/Rigid Transform  TranslationMethod=Cartesian  TranslationStandardOffset=0  TranslationLengthUnit=mm  TranslationStandardAxis=+Z  TranslationCartesianOffset=smiData.RigidTransform(4).translation  TranslationROffset=0  TranslationROffsetUnits=m  TranslationZOffset=0  TranslationZOffsetUnits=m  TranslationThetaOffset=0  TranslationThetaOffsetUnits=deg  RotationMethod=ArbitraryAxis  RotationAngleUnits=rad  RotationStandardAxis=+Z  RotationAngle=smiData.RigidTransform(4).angle  RotationArbitraryAxis=smiData.RigidTransform(4).axis  FollAlignAxisA=+X  BaseAlignAxisA=+Y  FollAlignAxisB=+Y  BaseAlignAxisB=+Z  RotationSequenceAxes=FollowerAxes  RotationSequence=XYX  RotationSequenceAngles=[0 0 0]  RotationSequenceAnglesUnits=deg  RotationMatrix=[1 0 0; 0 1 0; 0 0 1]
  F : PMIOPort  Side=Left
  connections:
  Transform/RConn1 -- F/RConn1
  Transform/LConn1 -- ReferenceFrame/RConn1 -- Solid/RConn1

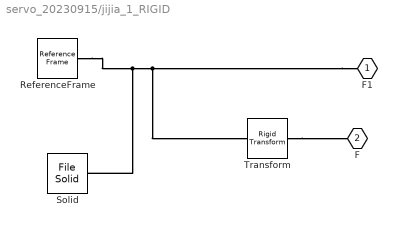
== system servo_20230915/jijia_1_RIGID ==
  ReferenceFrame : sm_lib/Frames and Transforms/Reference Frame
  Solid : sm_lib/Body Elements/File Solid  ExtGeomFileName=jijia_默认_sldprt.STEP  UnitType=FromFile  ExtGeomFileUnits=m  StepReaderType=HEX  ExportConvexHullGeometry=off  InertiaType=Custom  Mass=smiData.Solid(2).mass  MassUnits=kg  CenterOfMass=smiData.Solid(2).CoM  CenterOfMassUnits=mm  MomentsOfInertia=smiData.Solid(2).MoI  MomentsOfInertiaUnits=kg*mm^2  ProductsOfInertia=smiData.Solid(2).PoI  ProductsOfInertiaUnits=kg*mm^2  BasedOnType=Density  Density=1000  DensityUnits=kg/m^3  DoExposeReferenceFrame=on  SerializedFrames=<Frames/>  GraphicType=FromGeometry  MarkerShape=Sphere  MarkerSize=10  GraphicVisPropType=SimpleVisualProperties  GraphicDiffuseColor=smiData.Solid(2).color  GraphicSpecularColor=[0.5 0.5 0.5 1.0]  GraphicAmbientColor=[0.15 0.15 0.15 1.0]  GraphicEmissiveColor=[0.0 0.0 0.0 1.0]  GraphicShininess=75  GraphicOpacity=smiData.Solid(2).opacity
  Transform : sm_lib/Frames and Transforms/Rigid Transform  TranslationMethod=Cartesian  TranslationStandardOffset=0  TranslationLengthUnit=mm  TranslationStandardAxis=+Z  TranslationCartesianOffset=smiData.RigidTransform(1).translation  TranslationROffset=0  TranslationROffsetUnits=m  TranslationZOffset=0  TranslationZOffsetUnits=m  TranslationThetaOffset=0  TranslationThetaOffsetUnits=deg  RotationMethod=ArbitraryAxis  RotationAngleUnits=rad  RotationStandardAxis=+Z  RotationAngle=smiData.RigidTransform(1).angle  RotationArbitraryAxis=smiData.RigidTransform(1).axis  FollAlignAxisA=+X  BaseAlignAxisA=+Y  FollAlignAxisB=+Y  BaseAlignAxisB=+Z  RotationSequenceAxes=FollowerAxes  RotationSequence=XYX  RotationSequenceAngles=[0 0 0]  RotationSequenceAnglesUnits=deg  RotationMatrix=[1 0 0; 0 1 0; 0 0 1]
  F1 : PMIOPort  Side=Left
  F : PMIOPort  Port=2  Side=Right
  connections:
  Transform/RConn1 -- F/RConn1
  F1/RConn1 -- Transform/LConn1 -- ReferenceFrame/RConn1 -- Solid/RConn1

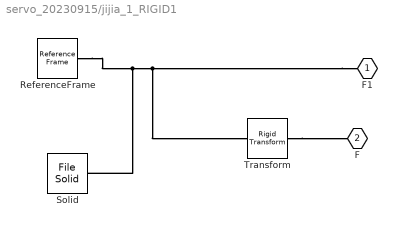
== system servo_20230915/jijia_1_RIGID1 ==
  ReferenceFrame : sm_lib/Frames and Transforms/Reference Frame
  Solid : sm_lib/Body Elements/File Solid  ExtGeomFileName=jijia_默认_sldprt.STEP  UnitType=FromFile  ExtGeomFileUnits=m  StepReaderType=HEX  ExportConvexHullGeometry=off  InertiaType=Custom  Mass=smiData.Solid(2).mass  MassUnits=kg  CenterOfMass=smiData.Solid(2).CoM  CenterOfMassUnits=mm  MomentsOfInertia=smiData.Solid(2).MoI  MomentsOfInertiaUnits=kg*mm^2  ProductsOfInertia=smiData.Solid(2).PoI  ProductsOfInertiaUnits=kg*mm^2  BasedOnType=Density  Density=1000  DensityUnits=kg/m^3  DoExposeReferenceFrame=on  SerializedFrames=<Frames/>  GraphicType=FromGeometry  MarkerShape=Sphere  MarkerSize=10  GraphicVisPropType=SimpleVisualProperties  GraphicDiffuseColor=[0.2 0.2 0.2]  GraphicSpecularColor=[0.5 0.5 0.5 1.0]  GraphicAmbientColor=[0.15 0.15 0.15 1.0]  GraphicEmissiveColor=[0.0 0.0 0.0 1.0]  GraphicShininess=75  GraphicOpacity=smiData.Solid(2).opacity
  Transform : sm_lib/Frames and Transforms/Rigid Transform  TranslationMethod=Cartesian  TranslationStandardOffset=0  TranslationLengthUnit=mm  TranslationStandardAxis=+Z  TranslationCartesianOffset=smiData.RigidTransform(1).translation  TranslationROffset=0  TranslationROffsetUnits=m  TranslationZOffset=0  TranslationZOffsetUnits=m  TranslationThetaOffset=0  TranslationThetaOffsetUnits=deg  RotationMethod=ArbitraryAxis  RotationAngleUnits=rad  RotationStandardAxis=+Z  RotationAngle=smiData.RigidTransform(1).angle  RotationArbitraryAxis=smiData.RigidTransform(1).axis  FollAlignAxisA=+X  BaseAlignAxisA=+Y  FollAlignAxisB=+Y  BaseAlignAxisB=+Z  RotationSequenceAxes=FollowerAxes  RotationSequence=XYX  RotationSequenceAngles=[0 0 0]  RotationSequenceAnglesUnits=deg  RotationMatrix=[1 0 0; 0 1 0; 0 0 1]
  F1 : PMIOPort  Side=Left
  F : PMIOPort  Port=2  Side=Right
  connections:
  Transform/RConn1 -- F/RConn1
  F1/RConn1 -- Transform/LConn1 -- ReferenceFrame/RConn1 -- Solid/RConn1
